simulink model "mixr1_v2_dev"  (R2026a)
settings: Solver=FixedStepAuto  StopTime=inf  FixedStep=0.05  EnableMultiTasking=on
undefined symbols (not defined in the file or in its folder): mixr1_bench, student_band, student_mode, student_pumpV, student_sp
(part 1 of 2)
settings Model: SimulationMode=external  ExtModeTrigDuration=2  Creator=Cyril Calo  LastModifiedBy=Cyril Calo
settings SolverCC: PositivePriorityOrder=on
settings OptimizationCC: MaxStackSize=200000
settings DebuggingCC: SubsystemReferenceDiagnosticForUnitTest=warning
settings HardwareCC: ProdBitPerLong=64.0  ProdLargestAtomicInteger=LongLong  ProdLargestAtomicFloat=Double  ProdHWDeviceType=ARM Compatible->ARM Cortex-A (64-bit)
settings RTWCC: SystemTargetFile=ert.tlc  HardwareBoard=Raspberry Pi (64bit)  TLCOptions="-aInlineSetEventsForThisBaseRateFcn=TLC_FALSE -aSuppressMultiTaskScheduler=TLC_FALSE  -aRateBasedStepFcn=0"  GenerateReport=on  CustomHeaderCode="#include \"act2_wrapper.h\""  CustomTerminator=act2_stop();  Toolchain=GNU GCC RPIUtils  BuildConfiguration=Faster Runs  LaunchReport=on  Description=Embedded Coder
settings CodeAppCC: MATLABSourceComments=on
settings ERTTargetCC: ExtModeTransport=2.0  DynamicArrayContainerType=coder::array  ERTCustomFileBanners=off  SupportContinuousTime=on  SupportNonInlinedSFcns=on  SupportVariableSizeSignals=on  ModelStepFunctionPrototypeControlCompliant=off

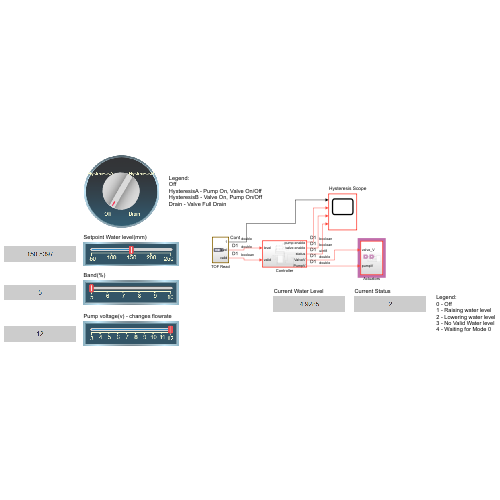
[thumbnail: Simulink's stored preview of the top-level diagram]
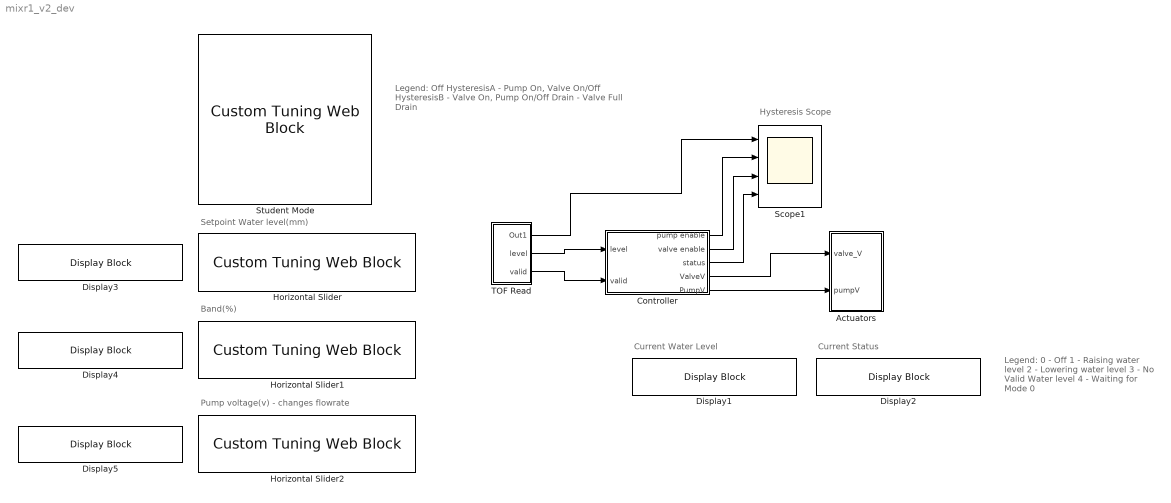
== system mixr1_v2_dev ==
  note: Current Water Level
  note: Legend:
      | Off
      | HysteresisA - Pump On, Valve On/Off
      | HysteresisB - Valve On, Pump On/Off
      | Drain - Valve Full Drain
  note: Setpoint Water level(mm)
  note: Band(%)
  note: Pump voltage(v) - changes flowrate
  note: Current Status
  note: Hysteresis Scope
  note: Legend:
      | 0 - Off
      | 1 - Raising water level
      | 2 - Lowering water level
      | 3 - No Valid Water level
      | 4 - Waiting for Mode 0
  Actuators : Subsystem
  Controller : Subsystem
  Display{1..5} (5 alike) : DisplayBlock  LabelPosition=Hide  Transparency=1  GridColor=[0.502, 0.502, 0.502]
  Horizontal Slider : CustomTuningWebBlock  LabelPosition=Hide  ShowInitialText=on  Configuration="{\"components\":[{\"name\":\"LinearScaleComponent\",\"settings\":{\"bounds\":{\"max\":250,\"min\":50,\"tickInterval\":\"auto\"},\"internalTickHeightScaleFactor\":0.5,\"labelColor\":[255,255,200],\"labelFont\":{\"font\":\"Arial\",\"fontSize\":12},\"labelOffset\":0.05,\"labelTransparency\":1,\"needleImage\":{\"size\":[596,842],\"src\":\"data:image\\/svg+xml;base64,PD94bWwgdmVyc2lvbj0iMS4wIiBlbmNvZGluZz0idXRmLTgiPz4NCjwhLS0gR2VuZXJhdG9yOiBBZG9iZSBJbGx1c3RyYXRvciAyNS4wLjAsIFNWRyBFeHBvcnQgUGx1Zy1JbiAuIFNWRyBWZXJzaW9uOiA2LjAwIEJ1aWxkIDApICAtLT4NCjxzdmcgdmVyc2lvbj0iMS4xIg0KCSBpZD0ic3ZnOCIgeG1sbnM6Y2M9Imh0dHA6Ly9jcmVhdGl2ZWNvbW1vbnMub3JnL25zIyIgeG1sbnM6ZGM9Imh0dHA6Ly9wdXJsLm9yZy9kYy9lbGVtZW50cy8xLjEvIiB4bWxuczppbmtzY2FwZT0iaHR0cDovL3d3dy5pbmtzY2FwZS5vcmcvbmFtZXNw ...(+2420 chars)\",\"srcOrientation\":\"Right\"},\"needleOffset\":[-0.8044596912521441,-0.0642123287671233],\"needleSize\":{\"height\":0.4337797619047619,\"width\":0.07668067226890757},\"position\":[0.2829861111111111,0.04398634453781513,0.9196428571428571,0.6088789682539683],\"referencePoint\":\"auto\",\"scaleColors\":[],\"scaleColorsSize\":0.2,\"scaleDirection\":\"LR\",\"showLabels\":1,\"showMinorTicks\":0,\"showSpanLine\":1,\"showTicks\":1,\"tickColor\":[252,252,197],\"tickTransparency\":1,\"valueBarColor\":[0,114,189],\"valueBarOffset\":-0.27,\"valueBarSize\":0.1,\"valueBarTransparency\":1}},{\"name\":\"BackgroundImageComponent\",\"settings\":{\"image\":{\"size\":[380,101],\"src\":\"data:image\\/svg+xml;base64,PHN2ZyB4bWxucz0iaHR0cDovL3d3dy53My5vcmcvMjAwMC9zdmciIHhtbG5zOnhsaW5rPSJodHRwOi8vd3d3LnczLm9yZy8xOTk5L3hsaW5rIiB2aWV3Qm94PSIwIDAgMzgwIDEwMSI+PGRlZnM+PHN0eWxlPi5jbHMtMXtmaWxsOiMwMDJiNDI7fS5jbHMtMntmaWxsOiM0MjcwODI7fS5jbHMtM3tmaWxsOnVybCgjcmFkaWFsLWdyYWRpZW50KTt9LmNscy00e2ZpbGw6I2M4YzhjODtzdHJva2U6IzAwMDt9PC9zdHlsZT48cmFkaWFsR3JhZGllbnQgaWQ9InJhZGlhbC1ncmFkaWVudCIgY3g9IjE5MCIgY3k9IjUwLjUiIHI9IjI2OS4yMSIgZ3JhZGllbnRVbml0cz0idXNlclNwYWNlT25Vc2UiPjxzdG9wIG9mZnNldD0iMC4wMSIgc3RvcC1jb2xvcj0iIzNlNGY1OCIvPjxzdG9wIG9mZnNldD0iMC4wNiIgc3RvcC1jb2xvcj0iIzQ0NTc2MSIvPjxzdG9wIG9mZnNldD0iMC4xNSIgc3RvcC1jb2xvcj0iIzU1NmE3NiIvPjxzdG9wIG9mZnNldD0iMC4yNSIgc3RvcC1jb2xvcj0iIzZkODg5NSIvPjxzdG9wIG9mZnNldD0iMC4zOCIgc3RvcC1jb2xvcj0iIzhmYjJjMyIvPjxzdG9wIG9mZnNldD0iMC41MiIgc3RvcC1jb2xvcj0iI2I2ZTRmYSIvPjxzdG9wIG9mZnNldD0iMSIgc3RvcC1jb2xvcj0iIzE1NDY1NyIvPjwvcmFkaWFsR3JhZGllbnQ+PC9kZWZzPjxnIGlkPSJmcmFtZSI+PGcgaWQ9IkxheWVyXzIiIGRhdGEtbmFtZT0iTGF5ZXIgMiI+PGcgaWQ9IkxheWVyXzEtMiIgZGF0YS1uYW1lPSJMYXllciAxLTIiPjxyZWN0IGlkPSJyZWN0MTAzNiIgY2xhc3M9ImNscy0xIiB4PSIxMSIgeT0iMTEiIHdpZHRoPSIzNTgiIGhlaWdodD0iNzkiLz48cGF0aCBpZD0icGF0aDEwMzgiIGNsYXNzPSJjbHMtMiIgZD0iTTgsOFY5M0gzNzJWOFpNMzY5LDkwSDExVjExSDM2OVoiLz48cGF0aCBpZD0icGF0aDEwNDAiIGNsYXNzPSJjbHMtMyIgZD0iTTAsMFYxMDFIMzgwVjBaTTM3Miw5M0g4VjhIMzcyWiIvPjwvZz48L2c+PC9nPjxnIGlkPSJ0cmFjayI+PHBhdGggaWQ9InJlY3QxNjExIiBjbGFzcz0iY2xzLTQiIGQ9Ik0zMy4zNywyNi41OUgzNDYuNjNjNCwwLDcuMjUsMi42LDcuMjUsNS44MWgwYzAsMy4yMS0zLjI1LDUuODItNy4yNSw1LjgySDMzLjM3Yy00LDAtNy4yNS0yLjYxLTcuMjUtNS44MmgwQzI2LjEyLDI5LjE5LDI5LjM3LDI2LjU5LDMzLjM3LDI2LjU5WiIvPjwvZz48L3N2Zz4=\",\"srcOrientation\":\"horizontal\"},\"position\":[0,0,1,1],\"scaleMode\":\"0\"}},{\"name\":\"ForegroundImageComponent\",\"settings\":{\"image\":{\"size\":[0,0],\"src\":\"default\",\"srcOrientation\":[]},\"isForeground\":1,\"position\":[0,0,1,1],\"scaleMode\":\"0\"}}],\"derived\":{\"blockParameters\":{\"ForegroundColor\":[0.9882352941176471,0.9882352941176471,0.7725490196078432],\"Limits\":{\"Max\":250,\"Min\":50,\"Ticks\":\"auto\"},\"ScaleColors\":[],\"ScaleDirection\":\"Clockwise\",\"ScaleMax\":250,\"ScaleMin\":50,\"TickInterval\":\"auto\",\"fixedAspectRatio\":\"on\"}},\"settings\":{\"BindingType\":\"param\",\"aspectRatio\":3.7777777777777777,\"backgroundColor\":[0,0,0,\"1\"],\"backgroundOffset\":0,\"backgroundOpacity\":1,\"fixedAspectRatio\":\"on\",\"foregroundColor\":[252,252,196],\"orientation\":\"horizontal\",\"showBackgroundColor\":false,\"value\":0,\"version\":\"R2023a\"},\"type\":\"LinearGauge\"}"
  Horizontal Slider1 : CustomTuningWebBlock  LabelPosition=Hide  ShowInitialText=on  Configuration="{\"components\":[{\"name\":\"LinearScaleComponent\",\"settings\":{\"bounds\":{\"max\":10,\"min\":5,\"tickInterval\":\"auto\"},\"internalTickHeightScaleFactor\":0.5,\"labelColor\":[255,255,200],\"labelFont\":{\"font\":\"Arial\",\"fontSize\":12},\"labelOffset\":0.05,\"labelTransparency\":1,\"needleImage\":{\"size\":[596,842],\"src\":\"data:image\\/svg+xml;base64,PD94bWwgdmVyc2lvbj0iMS4wIiBlbmNvZGluZz0idXRmLTgiPz4NCjwhLS0gR2VuZXJhdG9yOiBBZG9iZSBJbGx1c3RyYXRvciAyNS4wLjAsIFNWRyBFeHBvcnQgUGx1Zy1JbiAuIFNWRyBWZXJzaW9uOiA2LjAwIEJ1aWxkIDApICAtLT4NCjxzdmcgdmVyc2lvbj0iMS4xIg0KCSBpZD0ic3ZnOCIgeG1sbnM6Y2M9Imh0dHA6Ly9jcmVhdGl2ZWNvbW1vbnMub3JnL25zIyIgeG1sbnM6ZGM9Imh0dHA6Ly9wdXJsLm9yZy9kYy9lbGVtZW50cy8xLjEvIiB4bWxuczppbmtzY2FwZT0iaHR0cDovL3d3dy5pbmtzY2FwZS5vcmcvbmFtZXNw ...(+2420 chars)\",\"srcOrientation\":\"Right\"},\"needleOffset\":[-0.8044596912521441,-0.0642123287671233],\"needleSize\":{\"height\":0.4337797619047619,\"width\":0.07668067226890757},\"position\":[0.2829861111111111,0.04398634453781513,0.9196428571428571,0.6088789682539683],\"referencePoint\":\"auto\",\"scaleColors\":[],\"scaleColorsSize\":0.2,\"scaleDirection\":\"LR\",\"showLabels\":1,\"showMinorTicks\":0,\"showSpanLine\":1,\"showTicks\":1,\"tickColor\":[252,252,197],\"tickTransparency\":1,\"valueBarColor\":[0,114,189],\"valueBarOffset\":-0.27,\"valueBarSize\":0.1,\"valueBarTransparency\":1}},{\"name\":\"BackgroundImageComponent\",\"settings\":{\"image\":{\"size\":[380,101],\"src\":\"data:image\\/svg+xml;base64,PHN2ZyB4bWxucz0iaHR0cDovL3d3dy53My5vcmcvMjAwMC9zdmciIHhtbG5zOnhsaW5rPSJodHRwOi8vd3d3LnczLm9yZy8xOTk5L3hsaW5rIiB2aWV3Qm94PSIwIDAgMzgwIDEwMSI+PGRlZnM+PHN0eWxlPi5jbHMtMXtmaWxsOiMwMDJiNDI7fS5jbHMtMntmaWxsOiM0MjcwODI7fS5jbHMtM3tmaWxsOnVybCgjcmFkaWFsLWdyYWRpZW50KTt9LmNscy00e2ZpbGw6I2M4YzhjODtzdHJva2U6IzAwMDt9PC9zdHlsZT48cmFkaWFsR3JhZGllbnQgaWQ9InJhZGlhbC1ncmFkaWVudCIgY3g9IjE5MCIgY3k9IjUwLjUiIHI9IjI2OS4yMSIgZ3JhZGllbnRVbml0cz0idXNlclNwYWNlT25Vc2UiPjxzdG9wIG9mZnNldD0iMC4wMSIgc3RvcC1jb2xvcj0iIzNlNGY1OCIvPjxzdG9wIG9mZnNldD0iMC4wNiIgc3RvcC1jb2xvcj0iIzQ0NTc2MSIvPjxzdG9wIG9mZnNldD0iMC4xNSIgc3RvcC1jb2xvcj0iIzU1NmE3NiIvPjxzdG9wIG9mZnNldD0iMC4yNSIgc3RvcC1jb2xvcj0iIzZkODg5NSIvPjxzdG9wIG9mZnNldD0iMC4zOCIgc3RvcC1jb2xvcj0iIzhmYjJjMyIvPjxzdG9wIG9mZnNldD0iMC41MiIgc3RvcC1jb2xvcj0iI2I2ZTRmYSIvPjxzdG9wIG9mZnNldD0iMSIgc3RvcC1jb2xvcj0iIzE1NDY1NyIvPjwvcmFkaWFsR3JhZGllbnQ+PC9kZWZzPjxnIGlkPSJmcmFtZSI+PGcgaWQ9IkxheWVyXzIiIGRhdGEtbmFtZT0iTGF5ZXIgMiI+PGcgaWQ9IkxheWVyXzEtMiIgZGF0YS1uYW1lPSJMYXllciAxLTIiPjxyZWN0IGlkPSJyZWN0MTAzNiIgY2xhc3M9ImNscy0xIiB4PSIxMSIgeT0iMTEiIHdpZHRoPSIzNTgiIGhlaWdodD0iNzkiLz48cGF0aCBpZD0icGF0aDEwMzgiIGNsYXNzPSJjbHMtMiIgZD0iTTgsOFY5M0gzNzJWOFpNMzY5LDkwSDExVjExSDM2OVoiLz48cGF0aCBpZD0icGF0aDEwNDAiIGNsYXNzPSJjbHMtMyIgZD0iTTAsMFYxMDFIMzgwVjBaTTM3Miw5M0g4VjhIMzcyWiIvPjwvZz48L2c+PC9nPjxnIGlkPSJ0cmFjayI+PHBhdGggaWQ9InJlY3QxNjExIiBjbGFzcz0iY2xzLTQiIGQ9Ik0zMy4zNywyNi41OUgzNDYuNjNjNCwwLDcuMjUsMi42LDcuMjUsNS44MWgwYzAsMy4yMS0zLjI1LDUuODItNy4yNSw1LjgySDMzLjM3Yy00LDAtNy4yNS0yLjYxLTcuMjUtNS44MmgwQzI2LjEyLDI5LjE5LDI5LjM3LDI2LjU5LDMzLjM3LDI2LjU5WiIvPjwvZz48L3N2Zz4=\",\"srcOrientation\":\"horizontal\"},\"position\":[0,0,1,1],\"scaleMode\":\"0\"}},{\"name\":\"ForegroundImageComponent\",\"settings\":{\"image\":{\"size\":[0,0],\"src\":\"default\",\"srcOrientation\":[]},\"isForeground\":1,\"position\":[0,0,1,1],\"scaleMode\":\"0\"}}],\"derived\":{\"blockParameters\":{\"ForegroundColor\":[0.9882352941176471,0.9882352941176471,0.7725490196078432],\"Limits\":{\"Max\":10,\"Min\":5,\"Ticks\":\"auto\"},\"ScaleColors\":[],\"ScaleDirection\":\"Clockwise\",\"ScaleMax\":10,\"ScaleMin\":5,\"TickInterval\":\"auto\",\"fixedAspectRatio\":\"on\"}},\"settings\":{\"BindingType\":\"param\",\"aspectRatio\":3.7777777777777777,\"backgroundColor\":[0,0,0,\"1\"],\"backgroundOffset\":0,\"backgroundOpacity\":1,\"fixedAspectRatio\":\"on\",\"foregroundColor\":[252,252,196],\"orientation\":\"horizontal\",\"showBackgroundColor\":false,\"value\":0,\"version\":\"R2023a\"},\"type\":\"LinearGauge\"}"
  Horizontal Slider2 : CustomTuningWebBlock  LabelPosition=Hide  ShowInitialText=on  Configuration="{\"components\":[{\"name\":\"LinearScaleComponent\",\"settings\":{\"bounds\":{\"max\":12,\"min\":3,\"tickInterval\":\"auto\"},\"internalTickHeightScaleFactor\":0.5,\"labelColor\":[255,255,200],\"labelFont\":{\"font\":\"Arial\",\"fontSize\":12},\"labelOffset\":0.05,\"labelTransparency\":1,\"needleImage\":{\"size\":[596,842],\"src\":\"data:image\\/svg+xml;base64,PD94bWwgdmVyc2lvbj0iMS4wIiBlbmNvZGluZz0idXRmLTgiPz4NCjwhLS0gR2VuZXJhdG9yOiBBZG9iZSBJbGx1c3RyYXRvciAyNS4wLjAsIFNWRyBFeHBvcnQgUGx1Zy1JbiAuIFNWRyBWZXJzaW9uOiA2LjAwIEJ1aWxkIDApICAtLT4NCjxzdmcgdmVyc2lvbj0iMS4xIg0KCSBpZD0ic3ZnOCIgeG1sbnM6Y2M9Imh0dHA6Ly9jcmVhdGl2ZWNvbW1vbnMub3JnL25zIyIgeG1sbnM6ZGM9Imh0dHA6Ly9wdXJsLm9yZy9kYy9lbGVtZW50cy8xLjEvIiB4bWxuczppbmtzY2FwZT0iaHR0cDovL3d3dy5pbmtzY2FwZS5vcmcvbmFtZXNw ...(+2420 chars)\",\"srcOrientation\":\"Right\"},\"needleOffset\":[-0.8044596912521441,-0.0642123287671233],\"needleSize\":{\"height\":0.4337797619047619,\"width\":0.07668067226890757},\"position\":[0.2829861111111111,0.04398634453781513,0.9196428571428571,0.6088789682539683],\"referencePoint\":\"auto\",\"scaleColors\":[],\"scaleColorsSize\":0.2,\"scaleDirection\":\"LR\",\"showLabels\":1,\"showMinorTicks\":0,\"showSpanLine\":1,\"showTicks\":1,\"tickColor\":[252,252,197],\"tickTransparency\":1,\"valueBarColor\":[0,114,189],\"valueBarOffset\":-0.27,\"valueBarSize\":0.1,\"valueBarTransparency\":1}},{\"name\":\"BackgroundImageComponent\",\"settings\":{\"image\":{\"size\":[380,101],\"src\":\"data:image\\/svg+xml;base64,PHN2ZyB4bWxucz0iaHR0cDovL3d3dy53My5vcmcvMjAwMC9zdmciIHhtbG5zOnhsaW5rPSJodHRwOi8vd3d3LnczLm9yZy8xOTk5L3hsaW5rIiB2aWV3Qm94PSIwIDAgMzgwIDEwMSI+PGRlZnM+PHN0eWxlPi5jbHMtMXtmaWxsOiMwMDJiNDI7fS5jbHMtMntmaWxsOiM0MjcwODI7fS5jbHMtM3tmaWxsOnVybCgjcmFkaWFsLWdyYWRpZW50KTt9LmNscy00e2ZpbGw6I2M4YzhjODtzdHJva2U6IzAwMDt9PC9zdHlsZT48cmFkaWFsR3JhZGllbnQgaWQ9InJhZGlhbC1ncmFkaWVudCIgY3g9IjE5MCIgY3k9IjUwLjUiIHI9IjI2OS4yMSIgZ3JhZGllbnRVbml0cz0idXNlclNwYWNlT25Vc2UiPjxzdG9wIG9mZnNldD0iMC4wMSIgc3RvcC1jb2xvcj0iIzNlNGY1OCIvPjxzdG9wIG9mZnNldD0iMC4wNiIgc3RvcC1jb2xvcj0iIzQ0NTc2MSIvPjxzdG9wIG9mZnNldD0iMC4xNSIgc3RvcC1jb2xvcj0iIzU1NmE3NiIvPjxzdG9wIG9mZnNldD0iMC4yNSIgc3RvcC1jb2xvcj0iIzZkODg5NSIvPjxzdG9wIG9mZnNldD0iMC4zOCIgc3RvcC1jb2xvcj0iIzhmYjJjMyIvPjxzdG9wIG9mZnNldD0iMC41MiIgc3RvcC1jb2xvcj0iI2I2ZTRmYSIvPjxzdG9wIG9mZnNldD0iMSIgc3RvcC1jb2xvcj0iIzE1NDY1NyIvPjwvcmFkaWFsR3JhZGllbnQ+PC9kZWZzPjxnIGlkPSJmcmFtZSI+PGcgaWQ9IkxheWVyXzIiIGRhdGEtbmFtZT0iTGF5ZXIgMiI+PGcgaWQ9IkxheWVyXzEtMiIgZGF0YS1uYW1lPSJMYXllciAxLTIiPjxyZWN0IGlkPSJyZWN0MTAzNiIgY2xhc3M9ImNscy0xIiB4PSIxMSIgeT0iMTEiIHdpZHRoPSIzNTgiIGhlaWdodD0iNzkiLz48cGF0aCBpZD0icGF0aDEwMzgiIGNsYXNzPSJjbHMtMiIgZD0iTTgsOFY5M0gzNzJWOFpNMzY5LDkwSDExVjExSDM2OVoiLz48cGF0aCBpZD0icGF0aDEwNDAiIGNsYXNzPSJjbHMtMyIgZD0iTTAsMFYxMDFIMzgwVjBaTTM3Miw5M0g4VjhIMzcyWiIvPjwvZz48L2c+PC9nPjxnIGlkPSJ0cmFjayI+PHBhdGggaWQ9InJlY3QxNjExIiBjbGFzcz0iY2xzLTQiIGQ9Ik0zMy4zNywyNi41OUgzNDYuNjNjNCwwLDcuMjUsMi42LDcuMjUsNS44MWgwYzAsMy4yMS0zLjI1LDUuODItNy4yNSw1LjgySDMzLjM3Yy00LDAtNy4yNS0yLjYxLTcuMjUtNS44MmgwQzI2LjEyLDI5LjE5LDI5LjM3LDI2LjU5LDMzLjM3LDI2LjU5WiIvPjwvZz48L3N2Zz4=\",\"srcOrientation\":\"horizontal\"},\"position\":[0,0,1,1],\"scaleMode\":\"0\"}},{\"name\":\"ForegroundImageComponent\",\"settings\":{\"image\":{\"size\":[0,0],\"src\":\"default\",\"srcOrientation\":[]},\"isForeground\":1,\"position\":[0,0,1,1],\"scaleMode\":\"0\"}}],\"derived\":{\"blockParameters\":{\"ForegroundColor\":[0.9882352941176471,0.9882352941176471,0.7725490196078432],\"Limits\":{\"Max\":12,\"Min\":3,\"Ticks\":\"auto\"},\"ScaleColors\":[],\"ScaleDirection\":\"Clockwise\",\"ScaleMax\":12,\"ScaleMin\":3,\"TickInterval\":\"auto\",\"fixedAspectRatio\":\"on\"}},\"settings\":{\"BindingType\":\"param\",\"aspectRatio\":3.7777777777777777,\"backgroundColor\":[0,0,0,\"1\"],\"backgroundOffset\":0,\"backgroundOpacity\":1,\"fixedAspectRatio\":\"on\",\"foregroundColor\":[252,252,196],\"orientation\":\"horizontal\",\"showBackgroundColor\":false,\"value\":0,\"version\":\"R2023a\"},\"type\":\"LinearGauge\"}"
  Scope1 : Scope  NumInputPorts=4
      settings: ActiveDisplayYMinimum=-16.272808334060326  ActiveDisplayYMaximum=151.52170364309652
  Student Mode : CustomTuningWebBlock  LabelPosition=Hide  ShowInitialText=on  Configuration="{\"components\":[{\"name\":\"RotarySwitchComponent\",\"settings\":{\"arcAngle\":300,\"arcAngleOffset\":120,\"handle\":{\"size\":[150,150],\"src\":\"data:image\\/svg+xml;base64,PHN2ZyBpZD0iTGF5ZXJfMSIgZGF0YS1uYW1lPSJMYXllciAxIiB4bWxucz0iaHR0cDovL3d3dy53My5vcmcvMjAwMC9zdmciIHhtbG5zOnhsaW5rPSJodHRwOi8vd3d3LnczLm9yZy8xOTk5L3hsaW5rIiB2aWV3Qm94PSIwIDAgMTIxIDEyMSI+PGRlZnM+PHN0eWxlPi5jbHMtMXtmaWxsOnVybCgjbGluZWFyLWdyYWRpZW50KTt9LmNscy0yLC5jbHMtM3tmaWxsOiNkMWQxZDE7fS5jbHMtM3tzdHJva2U6I2I3YjdiNztzdHJva2UtbWl0ZXJsaW1pdDoxMDtzdHJva2Utd2lkdGg6MC4yNXB4O30uY2xzLTR7ZmlsbDojZjMwMDAwO30uY2xzLTV7ZmlsbDojZjIxNzY3O308L3N0eWxlPjxsaW5lYXJHcmFkaWVudCBpZD0ibGluZWFyLWdyYWRpZW50IiB4MT0iNjAuNSIgeTE9IjEyMC41IiB4Mj0iNjAuNSIgeTI9IjAuNSIgZ3JhZGllbnRVbml0cz0idXNlclNwYWNlT25Vc2UiPjxzdG9wIG9mZnNldD0iMCIgc3RvcC1jb2xvcj0iI2QxZDFkMSIvPjxzdG9wIG9mZnNldD0iMC4xIiBzdG9wLWNvbG9yPSIjY2VjZWNlIi8+PHN0b3Agb2Zmc2V0PSIwLjE5IiBzdG9wLWNvbG9yPSIjYzNjM2MzIi8+PHN0b3Agb2Zmc2V0PSIwLjI4IiBzdG9wLWNvbG9yPSIjYjFiMWIxIi8+PHN0b3Agb2Zmc2V0PSIwLjM2IiBzdG9wLWNvbG9yPSIjOTg5ODk4Ii8+PHN0b3Agb2Zmc2V0PSIwLjQ0IiBzdG9wLWNvbG9yPSIjNzg3ODc4Ii8+PHN0b3Agb2Zmc2V0PSIwLjQ2IiBzdG9wLWNvbG9yPSIjNmI2YjZiIi8+PHN0b3Agb2Zmc2V0PSIwLjU0IiBzdG9wLWNvbG9yPSIjNmI2YjZiIi8+PHN0b3Agb2Zmc2V0PSIwLjU2IiBzdG9wLWNvbG9yPSIjNzY3Njc2Ii8+PHN0b3Agb2Zmc2V0PSIwLjY0IiBzdG9wLWNvbG9yPSIjOTc5Nzk3Ii8+PHN0b3Agb2Zmc2V0PSIwLjcyIiBzdG9wLWNvbG9yPSIjYjBiMGIwIi8+PHN0b3Agb2Zmc2V0PSIwLjgxIiBzdG9wLWNvbG9yPSIjYzNjM2MzIi8+PHN0b3Agb2Zmc2V0PSIwLjkiIHN0b3AtY29sb3I9IiNjZGNkY2QiLz48c3RvcCBvZmZzZXQ9IjEiIHN0b3AtY29sb3I9IiNkMWQxZDEiLz48L2xpbmVhckdyYWRpZW50PjwvZGVmcz48Y2lyY2xlIGNsYXNzPSJjbHMtMSIgY3g9IjYwLjUiIGN5PSI2MC41IiByPSI2MCIvPjxwYXRoIGNsYXNzPSJjbHMtMiIgZD0iTTYwLjUsMUE1OS41LDU5LjUsMCwxLDEsMSw2MC41LDU5LjU3LDU5LjU3LDAsMCwxLDYwLjUsMW0wLTFBNjAuNSw2MC41LDAsMSwwLDEyMSw2MC41LDYwLjUsNjAuNSwwLDAsMCw2MC41LDBaIi8+PHJlY3QgY2xhc3M9ImNscy0zIiB4PSIwLjUiIHk9IjUxLjUiIHdpZHRoPSIxMjAiIGhlaWdodD0iMTgiIHJ4PSIzLjA0Ii8+PHJlY3QgY2xhc3M9ImNscy00IiB4PSI1Ljc1IiB5PSI1OC43NSIgd2lkdGg9IjE2IiBoZWlnaHQ9IjMiLz48cGF0aCBjbGFzcz0iY2xzLTUiIGQ9Ik0yMS4yNSw1OS4yNXYyaC0xNXYtMmgxNW0xLTFoLTE3djRoMTd2LTRaIi8+PC9zdmc+\"},\"handleOffset\":[0,0],\"handleOrientation\":180,\"handlePosition\":[0,0,1,1],\"handleSize\":{\"height\":0.5,\"width\":0.5},\"labelRadius\":0.36,\"position\":[0,0,1,1],\"states\":[{\"Label\":{\"color\":[0,0,0,1],\"icon\":{\"size\":[0,0],\"src\":[],\"srcOrientation\":\"Right\"},\"iconOffset\":0,\"iconPlacement\":\"left\",\"opacity\":1,\"position\":[0.7345552884615385,0.6796274038461538],\"show\":true,\"text\":{\"content\":\"Off\",\"font\":\"Helvetica\"}},\"Value\":0},{\"Label\":{\"color\":[0,0,0,1],\"icon\":{\"size\":[0,0],\"src\":[],\"srcOrientation\":\"Right\"},\"iconOffset\":0,\"iconPlacement\":\"left\",\"opacity\":1,\"position\":[0.35757211538461536,0.7603966346153846],\"show\":true,\"text\":{\"content\":\"HysteresisA\",\"font\":\"Helvetica\"}},\"Value\":1},{\"Label\":{\"color\":[0,0,0,1],\"icon\":{\"size\":[0,0],\"src\":[],\"srcOrientation\":\"Right\"},\"iconOffset\":0,\"iconPlacement\":\"left\",\"opacity\":1,\"position\":[0.09603365384615385,0.46033653846153844],\"show\":true,\"text\":{\"content\":\"HysteresisB\",\"font\":\"Helvetica\"}},\"Value\":2},{\"Label\":{\"color\":[0,0,0,1],\"icon\":{\"size\":[0,0],\"src\":[],\"srcOrientation\":\"Right\"},\"iconOffset\":0,\"iconPlacement\":\"left\",\"opacity\":1,\"position\":[0.09603365384615385,0.46033653846153844],\"show\":true,\"text\":{\"content\":\"Drain\",\"font\":\"Helvetica\"}},\"Value\":3}],\"tickRadius\":0.32}},{\"name\":\"BackgroundImageComponent\",\"settings\":{\"image\":{\"size\":[155,150],\"src\":\"data:image\\/svg+xml;base64,PD94bWwgdmVyc2lvbj0iMS4wIiBlbmNvZGluZz0idXRmLTgiPz4NCjwhLS0gR2VuZXJhdG9yOiBBZG9iZSBJbGx1c3RyYXRvciAyNS4wLjAsIFNWRyBFeHBvcnQgUGx1Zy1JbiAuIFNWRyBWZXJzaW9uOiA2LjAwIEJ1aWxkIDApICAtLT4NCjxzdmcgdmVyc2lvbj0iMS4xIg0KCSBpZD0iTGF5ZXJfMl8xXyIgeG1sbnM6Y2M9Imh0dHA6Ly9jcmVhdGl2ZWNvbW1vbnMub3JnL25zIyIgeG1sbnM6ZGM9Imh0dHA6Ly9wdXJsLm9yZy9kYy9lbGVtZW50cy8xLjEvIiB4bWxuczppbmtzY2FwZT0iaHR0cDovL3d3dy5pbmtzY2FwZS5vcmcv ...(+4184 chars)\",\"srcOrientation\":\"Right\"},\"position\":[0,0,1,1],\"scaleMode\":\"0\"}},{\"name\":\"ForegroundImageComponent\",\"settings\":{\"image\":{\"size\":[0,0],\"src\":\"default\",\"srcOrientation\":[]},\"isForeground\":1,\"position\":[0,0,1,1],\"scaleMode\":\"0\"}}],\"derived\":{\"blockParameters\":{\"ForegroundColor\":[0.9882352941176471,0.9882352941176471,0.7725490196078432],\"States\":[{\"Label\":{\"color\":[0,0,0,1],\"icon\":{\"size\":[0,0],\"src\":[],\"srcOrientation\":\"Right\"},\"iconOffset\":0,\"iconPlacement\":\"left\",\"opacity\":1,\"position\":[0.7345552884615385,0.6796274038461538],\"show\":true,\"text\":{\"content\":\"Off\",\"font\":\"Helvetica\"}},\"Value\":0},{\"Label\":{\"color\":[0,0,0,1],\"icon\":{\"size\":[0,0],\"src\":[],\"srcOrientation\":\"Right\"},\"iconOffset\":0,\"iconPlacement\":\"left\",\"opacity\":1,\"position\":[0.35757211538461536,0.7603966346153846],\"show\":true,\"text\":{\"content\":\"HysteresisA\",\"font\":\"Helvetica\"}},\"Value\":1},{\"Label\":{\"color\":[0,0,0,1],\"icon\":{\"size\":[0,0],\"src\":[],\"srcOrientation\":\"Right\"},\"iconOffset\":0,\"iconPlacement\":\"left\",\"opacity\":1,\"position\":[0.09603365384615385,0.46033653846153844],\"show\":true,\"text\":{\"content\":\"HysteresisB\",\"font\":\"Helvetica\"}},\"Value\":2},{\"Label\":{\"color\":[0,0,0,1],\"icon\":{\"size\":[0,0],\"src\":[],\"srcOrientation\":\"Right\"},\"iconOffset\":0,\"iconPlacement\":\"left\",\"opacity\":1,\"position\":[0.09603365384615385,0.46033653846153844],\"show\":true,\"text\":{\"content\":\"Drain\",\"font\":\"Helvetica\"}},\"Value\":3}],\"StatesJSON\":[{\"Label\":\"Off\",\"Value\":0},{\"Label\":\"HysteresisA\",\"Value\":1},{\"Label\":\"HysteresisB\",\"Value\":2},{\"Label\":\"Drain\",\"Value\":3}],\"enumDataType\":\"\",\"fixedAspectRatio\":\"off\",\"useEnumDataType\":false}},\"settings\":{\"BindingType\":\"param\",\"backgroundColor\":[0,0,255,\"1\"],\"backgroundOffset\":1,\"fixedAspectRatio\":\"off\",\"image\":{\"size\":[150,150],\"src\":\"data:image\\/svg+xml;base64,PD94bWwgdmVyc2lvbj0iMS4wIiBlbmNvZGluZz0iVVRGLTgiIHN0YW5kYWxvbmU9Im5vIj8+CjwhLS0gR2VuZXJhdG9yOiBBZG9iZSBJbGx1c3RyYXRvciAxOS4yLjEsIFNWRyBFeHBvcnQgUGx1Zy1JbiAuIFNWRyBWZXJzaW9uOiA2LjAwIEJ1aWxkIDApICAtLT4KCjxzdmcKICAgeG1sbnM6ZGM9Imh0dHA6Ly9wdXJsLm9yZy9kYy9lbGVtZW50cy8xLjEvIgogICB4bWxuczpjYz0iaHR0cDovL2NyZWF0aXZlY29tbW9ucy5vcmcvbnMjIgogICB4bWxuczpyZGY9Imh0dHA6Ly93d3cudzMub3JnLzE5OTkvMDIvMjItcmRmLXN5bnRh ...(+9660 chars)\"},\"showBackgroundColor\":false,\"variant\":\"rotarySwitch\",\"version\":\"R2023a\"},\"type\":\"RotarySwitch\"}"
  TOF Read : Subsystem
  wires:
  Controller/1(pump enable) -> Scope1/2
  Controller/2(valve enable) -> Scope1/3
  Controller/3(status) -> Scope1/4
  TOF Read/1(Out1) -> Scope1/1
  TOF Read/2(level) -> Controller/1(level)
  TOF Read/3(valid) -> Controller/2(valid)
  Controller/4(ValveV) -> Actuators/1(valve_V)
  Controller/5(PumpV) -> Actuators/2(pumpV)

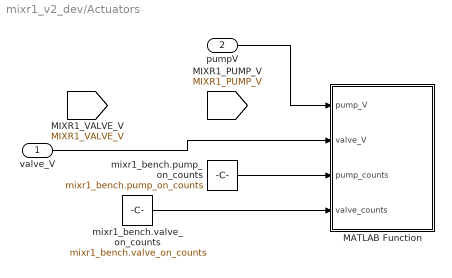
== system mixr1_v2_dev/Actuators ==
  valve_V : Inport
  pumpV : Inport  Port=2
  MATLAB Function : MATLAB Function  TreatAsAtomicUnit=on
  mixr1_bench.pump_on_counts : Constant  Value=mixr1_bench.pump_on_counts
  mixr1_bench.valve_on_counts : Constant  Value=mixr1_bench.valve_on_counts
  wires:
  mixr1_bench.pump_on_counts/1 -> MATLAB Function/3(pump_counts)
  mixr1_bench.valve_on_counts/1 -> MATLAB Function/4(valve_counts)
  valve_V/1 -> MATLAB Function/2(valve_V)
  pumpV/1 -> MATLAB Function/1(pump_V)

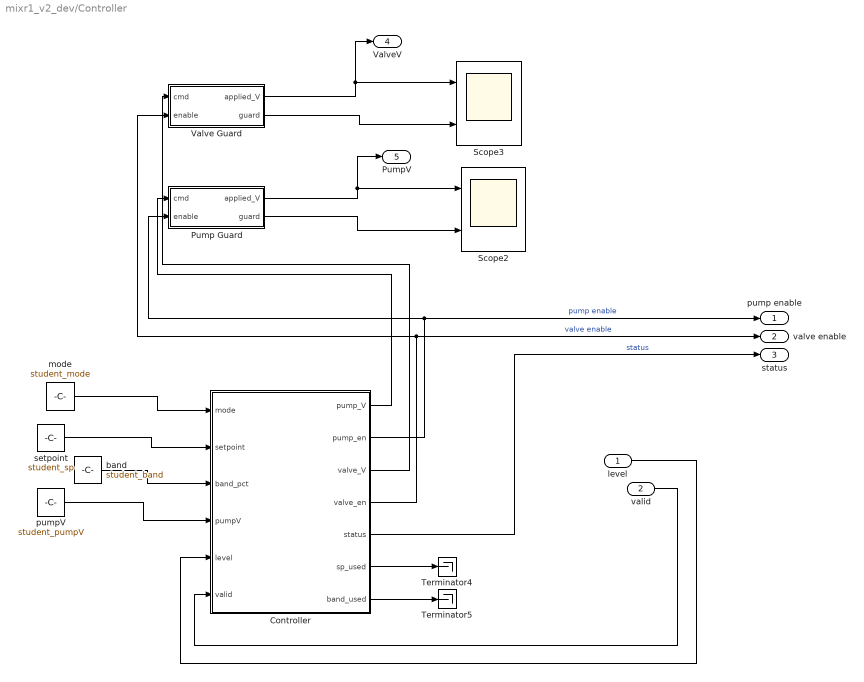
== system mixr1_v2_dev/Controller ==
  level : Inport
  valid : Inport  Port=2
  Controller : Subsystem
  Pump Guard : Subsystem
  Scope2 : Scope  NumInputPorts=2
      settings: ActiveDisplayYMinimum=-0.74999999999999978  ActiveDisplayYMaximum=6.75  DataLoggingVariableName=ScopeData2
  Scope3 : Scope  NumInputPorts=2
      settings: ActiveDisplayYMinimum=-0.74999999999999978  ActiveDisplayYMaximum=6.75  DataLoggingVariableName=ScopeData3
  Terminator4 : Terminator
  Terminator5 : Terminator
  Valve Guard : Subsystem
  band : Constant  Value=student_band
  mode : Constant  Value=student_mode
  pumpV : Constant  Value=student_pumpV
  setpoint : Constant  Value=student_sp
  pump enable : Outport
  valve enable : Outport  Port=2
  status : Outport  Port=3
  ValveV : Outport  Port=4
  PumpV : Outport  Port=5
  wires:
  Controller/4(valve_en) -> valve enable/1, Valve Guard/2(enable)  "valve enable"
  mode/1 -> Controller/1(mode)
  pumpV/1 -> Controller/4(pumpV)
  level/1 -> Controller/5(level)
  Controller/2(pump_en) -> pump enable/1, Pump Guard/2(enable)  "pump enable"
  Valve Guard/1(applied_V) -> ValveV/1, Scope3/1
  Controller/1(pump_V) -> Pump Guard/1(cmd)
  setpoint/1 -> Controller/2(setpoint)
  Pump Guard/1(applied_V) -> PumpV/1, Scope2/1
  Pump Guard/2(guard) -> Scope2/2
  band/1 -> Controller/3(band_pct)
  Controller/7(band_used) -> Terminator5/1
  Controller/3(valve_V) -> Valve Guard/1(cmd)
  Controller/6(sp_used) -> Terminator4/1
  Valve Guard/2(guard) -> Scope3/2
  Controller/5(status) -> status/1  "status"
  valid/1 -> Controller/6(valid)

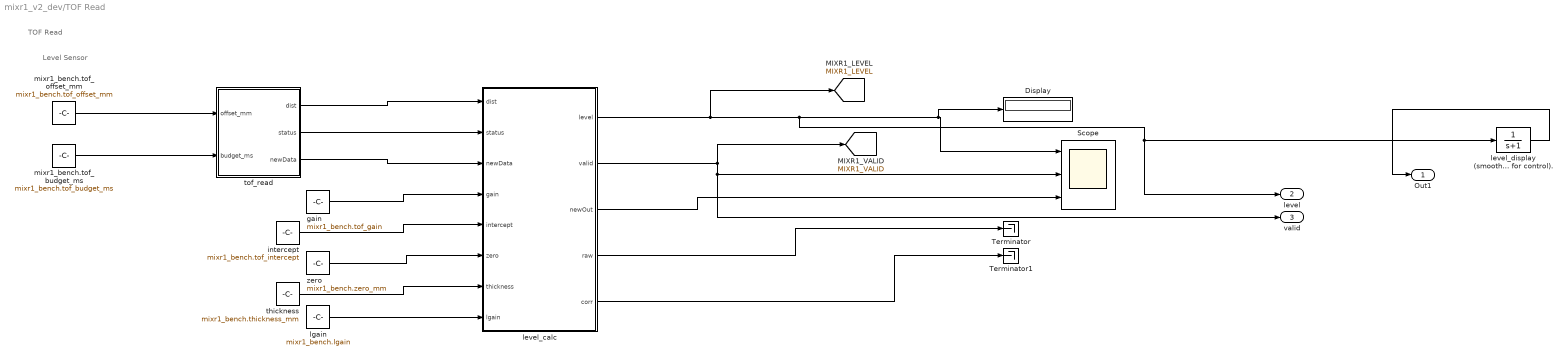
== system mixr1_v2_dev/TOF Read ==
  note: TOF Read
  note: Level Sensor
  Display : Display
  Scope : Scope  NumInputPorts=3
      settings: ActiveDisplayYMinimum=-14.994495697222678  ActiveDisplayYMaximum=154.35862672760038
  Terminator : Terminator
  Terminator1 : Terminator
  gain : Constant  Value=mixr1_bench.tof_gain
  intercept : Constant  Value=mixr1_bench.tof_intercept
  level_calc : MATLAB Function  TreatAsAtomicUnit=on
  "level_display (smoothed, display only — not used for control)." : TransferFcn  Denominator=[1 1]
  lgain : Constant  Value=mixr1_bench.lgain
  mixr1_bench.tof_budget_ms : Constant  Value=mixr1_bench.tof_budget_ms
  mixr1_bench.tof_offset_mm : Constant  Value=mixr1_bench.tof_offset_mm
  thickness : Constant  Value=mixr1_bench.thickness_mm
  tof_read : MATLAB Function  TreatAsAtomicUnit=on
  zero : Constant  Value=mixr1_bench.zero_mm
  Out1 : Outport
  level : Outport  Port=2
  valid : Outport  Port=3
  tag scope: MIXR1_LEVEL=global, MIXR1_VALID=global
  wires:
  mixr1_bench.tof_budget_ms/1 -> tof_read/2(budget_ms)
  mixr1_bench.tof_offset_mm/1 -> tof_read/1(offset_mm)
  level_calc/2(valid) -> valid/1, Scope/2, [MIXR1_VALID]
  level_calc/1(level) -> level/1, "level_display (smoothed, display only — not used for control)."/1, Scope/1, Display/1, [MIXR1_LEVEL]
  zero/1 -> level_calc/6(zero)
  lgain/1 -> level_calc/8(lgain)
  thickness/1 -> level_calc/7(thickness)
  gain/1 -> level_calc/4(gain)
  level_calc/5(corr) -> Terminator1/1
  "level_display (smoothed, display only — not used for control)."/1 -> Out1/1
  intercept/1 -> level_calc/5(intercept)
  tof_read/1(dist) -> level_calc/1(dist)
  tof_read/2(status) -> level_calc/2(status)
  tof_read/3(newData) -> level_calc/3(newData)
  level_calc/3(newOut) -> Scope/3
  level_calc/4(raw) -> Terminator/1

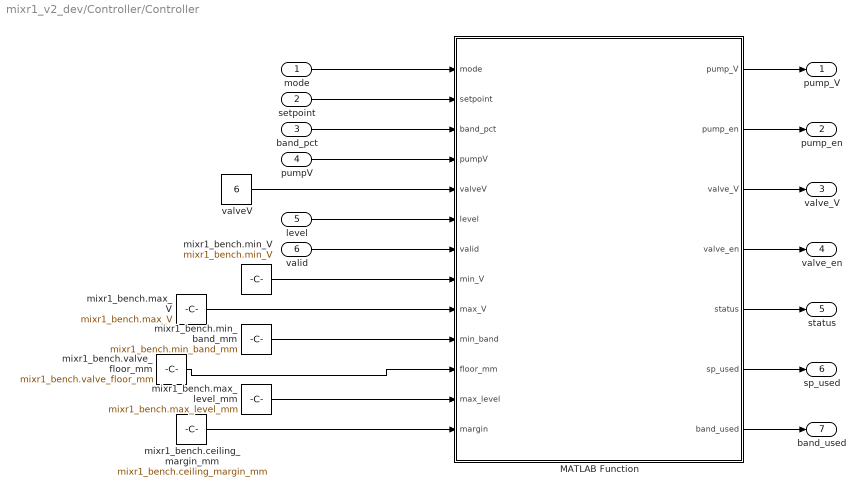
== system mixr1_v2_dev/Controller/Controller ==
  mode : Inport
  setpoint : Inport  Port=2
  band_pct : Inport  Port=3
  pumpV : Inport  Port=4
  level : Inport  Port=5
  valid : Inport  Port=6
  MATLAB Function : MATLAB Function  TreatAsAtomicUnit=on
  mixr1_bench.ceiling_margin_mm : Constant  Value=mixr1_bench.ceiling_margin_mm
  mixr1_bench.max_V : Constant  Value=mixr1_bench.max_V
  mixr1_bench.max_level_mm : Constant  Value=mixr1_bench.max_level_mm
  mixr1_bench.min_V : Constant  Value=mixr1_bench.min_V
  mixr1_bench.min_band_mm : Constant  Value=mixr1_bench.min_band_mm
  mixr1_bench.valve_floor_mm : Constant  Value=mixr1_bench.valve_floor_mm
  valveV : Constant  Value=6
  pump_V : Outport
  pump_en : Outport  Port=2
  valve_V : Outport  Port=3
  valve_en : Outport  Port=4
  status : Outport  Port=5
  sp_used : Outport  Port=6
  band_used : Outport  Port=7
  wires:
  mode/1 -> MATLAB Function/1(mode)
  setpoint/1 -> MATLAB Function/2(setpoint)
  band_pct/1 -> MATLAB Function/3(band_pct)
  pumpV/1 -> MATLAB Function/4(pumpV)
  valveV/1 -> MATLAB Function/5(valveV)
  level/1 -> MATLAB Function/6(level)
  valid/1 -> MATLAB Function/7(valid)
  mixr1_bench.min_V/1 -> MATLAB Function/8(min_V)
  mixr1_bench.max_V/1 -> MATLAB Function/9(max_V)
  mixr1_bench.min_band_mm/1 -> MATLAB Function/10(min_band)
  mixr1_bench.valve_floor_mm/1 -> MATLAB Function/11(floor_mm)
  mixr1_bench.max_level_mm/1 -> MATLAB Function/12(max_level)
  mixr1_bench.ceiling_margin_mm/1 -> MATLAB Function/13(margin)
  MATLAB Function/1(pump_V) -> pump_V/1
  MATLAB Function/2(pump_en) -> pump_en/1
  MATLAB Function/3(valve_V) -> valve_V/1
  MATLAB Function/4(valve_en) -> valve_en/1
  MATLAB Function/5(status) -> status/1
  MATLAB Function/6(sp_used) -> sp_used/1
  MATLAB Function/7(band_used) -> band_used/1

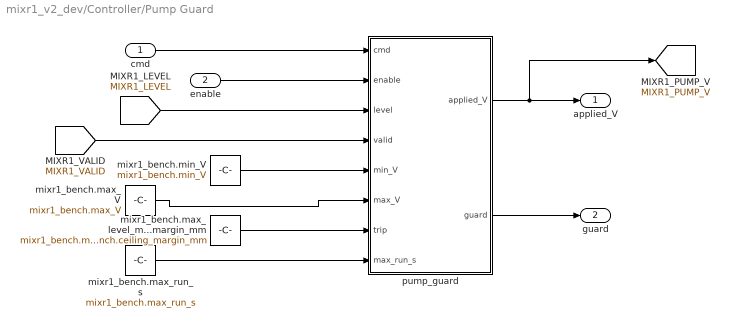
== system mixr1_v2_dev/Controller/Pump Guard ==
  cmd : Inport
  enable : Inport  Port=2
  mixr1_bench.max_V : Constant  Value=mixr1_bench.max_V
  mixr1_bench.max_level_mm - mixr1_bench.ceiling_margin_mm : Constant  Value=mixr1_bench.max_level_mm - mixr1_bench.ceiling_margin_mm
  mixr1_bench.max_run_s : Constant  Value=mixr1_bench.max_run_s
  mixr1_bench.min_V : Constant  Value=mixr1_bench.min_V
  pump_guard : MATLAB Function  TreatAsAtomicUnit=on
  applied_V : Outport
  guard : Outport  Port=2
  tag scope: MIXR1_PUMP_V=global
  wires:
  mixr1_bench.min_V/1 -> pump_guard/5(min_V)
  mixr1_bench.max_V/1 -> pump_guard/6(max_V)
  mixr1_bench.max_run_s/1 -> pump_guard/8(max_run_s)
  mixr1_bench.max_level_mm - mixr1_bench.ceiling_margin_mm/1 -> pump_guard/7(trip)
  [MIXR1_LEVEL] -> pump_guard/3(level)
  [MIXR1_VALID] -> pump_guard/4(valid)
  cmd/1 -> pump_guard/1(cmd)
  enable/1 -> pump_guard/2(enable)
  pump_guard/1(applied_V) -> [MIXR1_PUMP_V], applied_V/1
  pump_guard/2(guard) -> guard/1
